simulink model "SSB-SC Modulation and demodulation"  (R2025a)
settings: Solver=VariableStepAuto  StartTime=0.0  StopTime=10.0  RelTol=1e-3
libraries: dspsrcs4 x5, dspfdesign x1
settings Model: Creator=Aman  LastModifiedBy=Aman

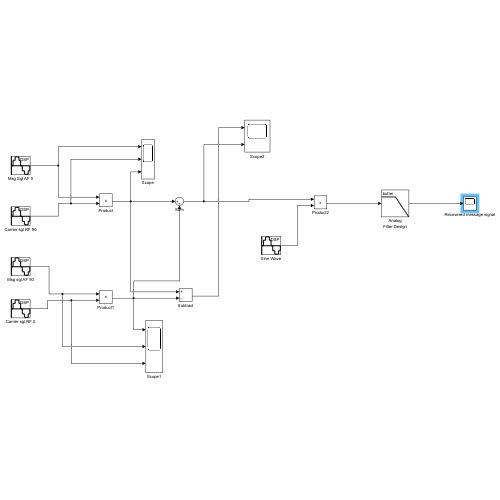
[thumbnail: Simulink's stored preview of the top-level diagram]
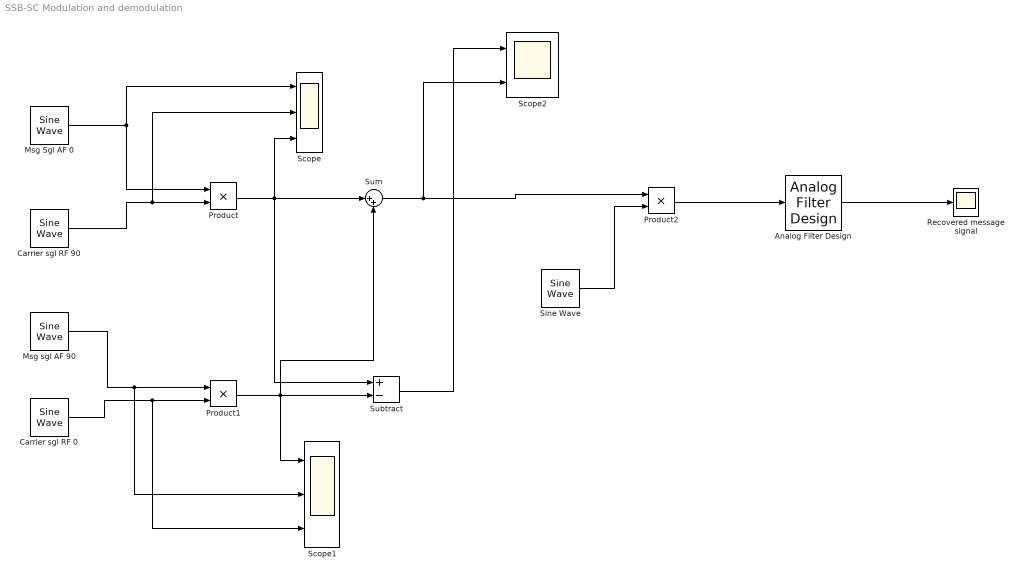
== system SSB-SC Modulation and demodulation ==
  Analog Filter Design : dspfdesign/Analog Filter Design  method=Butterworth  filttype=Lowpass  N=8  Wlo=2*pi*20  Whi=80  Rp=2  Rs=40
  Carrier sgl RF 0 : dspsrcs4/Sine Wave  Amplitude=1  Frequency=20  Phase=0  SampleMode=Discrete  OutComplex=Real  CompMethod=Trigonometric fcn  TableSize=Speed  SampleTime=1/1000  SamplesPerFrame=1  ResetState=Restart at time zero  OutputFrames=off  dataType=double  wordLen=16  udDataType=sfix(16)  fracBitsMode=Best precision  numFracBits=15  OutDataTypeStr=double  LastOutDataTypeStr=double
  Carrier sgl RF 90 : dspsrcs4/Sine Wave  Amplitude=1  Frequency=20  Phase=pi/2  SampleMode=Discrete  OutComplex=Real  CompMethod=Trigonometric fcn  TableSize=Speed  SampleTime=1/1000  SamplesPerFrame=1  ResetState=Restart at time zero  OutputFrames=off  dataType=double  wordLen=16  udDataType=sfix(16)  fracBitsMode=Best precision  numFracBits=15  OutDataTypeStr=double  LastOutDataTypeStr=double
  Msg Sgl AF 0 : dspsrcs4/Sine Wave  Amplitude=1  Frequency=2  Phase=0  SampleMode=Discrete  OutComplex=Real  CompMethod=Trigonometric fcn  TableSize=Speed  SampleTime=1/1000  SamplesPerFrame=1  ResetState=Restart at time zero  OutputFrames=off  dataType=double  wordLen=16  udDataType=sfix(16)  fracBitsMode=Best precision  numFracBits=15  OutDataTypeStr=double  LastOutDataTypeStr=double
  Msg sgl AF 90 : dspsrcs4/Sine Wave  Amplitude=1  Frequency=2  Phase=pi/2  SampleMode=Discrete  OutComplex=Real  CompMethod=Trigonometric fcn  TableSize=Speed  SampleTime=1/1000  SamplesPerFrame=1  ResetState=Restart at time zero  OutputFrames=off  dataType=double  wordLen=16  udDataType=sfix(16)  fracBitsMode=Best precision  numFracBits=15  OutDataTypeStr=double  LastOutDataTypeStr=double
  Product : Product
  Product1 : Product
  Product2 : Product
  Recovered message signal : Scope
      settings: ActiveDisplayYMinimum=-0.63459775711519928  ActiveDisplayYMaximum=0.7121128481653225  DataLoggingVariableName=ScopeData3
  Scope : Scope  NumInputPorts=3
      settings: ActiveDisplayYMinimum=-1.25  ActiveDisplayYMaximum=1.25
  Scope1 : Scope  NumInputPorts=3
      settings: ActiveDisplayYMinimum=-1.2333760829446874  ActiveDisplayYMaximum=1.2333760829446865  DataLoggingVariableName=ScopeData2
  Scope2 : Scope  NumInputPorts=2
      settings: ActiveDisplayYMinimum=-2.2089073634355492  ActiveDisplayYMaximum=1.0110506952824061
  Sine Wave : dspsrcs4/Sine Wave  Amplitude=1  Frequency=20  Phase=0  SampleMode=Discrete  OutComplex=Real  CompMethod=Trigonometric fcn  TableSize=Speed  SampleTime=1/1000  SamplesPerFrame=1  ResetState=Restart at time zero  OutputFrames=off  dataType=double  wordLen=16  udDataType=sfix(16)  fracBitsMode=Best precision  numFracBits=15  OutDataTypeStr=double  LastOutDataTypeStr=double
  Subtract : Sum  Inputs=+-
  Sum : Sum  Inputs=|++
  wires:
  Msg Sgl AF 0/1 -> Product/1, Scope/1
  Carrier sgl RF 90/1 -> Scope/2, Product/2
  Product/1 -> Subtract/1, Scope/3, Sum/1
  Msg sgl AF 90/1 -> Scope1/2, Product1/1
  Carrier sgl RF 0/1 -> Scope1/3, Product1/2
  Product1/1 -> Sum/2, Subtract/2, Scope1/1
  Sum/1 -> Scope2/2, Product2/1
  Product2/1 -> Analog Filter Design/1
  Analog Filter Design/1 -> Recovered message signal/1
  Sine Wave/1 -> Product2/2
  Subtract/1 -> Scope2/1
